simulink model "plant_block"  (R2025b)
settings: Solver=VariableStepAuto  StartTime=0.0  StopTime=10.0  RelTol=1e-3
undefined symbols (not defined in the file): auv
settings Model: Creator=Heisenberg  LastModifiedBy=Heisenberg

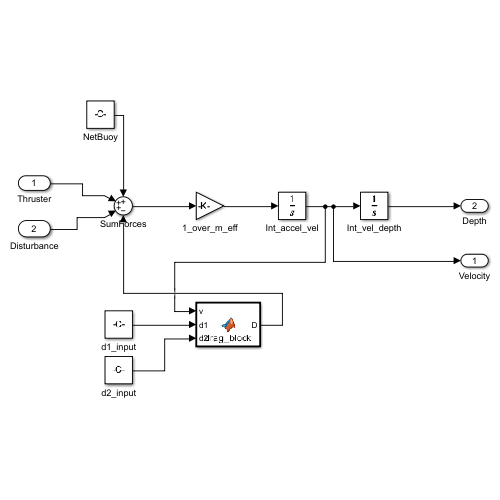
[thumbnail: Simulink's stored preview of the top-level diagram]
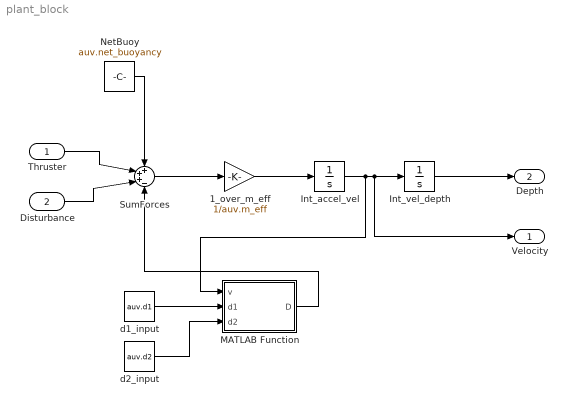
== system plant_block ==
  Thruster : Inport
  Disturbance : Inport  Port=2
  1_over_m_eff : Gain  Gain=1/auv.m_eff
  Int_accel_vel : Integrator
  Int_vel_depth : Integrator
  MATLAB Function : MATLAB Function  TreatAsAtomicUnit=on
  NetBuoy : Constant  Value=auv.net_buoyancy
  SumForces : Sum  Inputs=+++-
  d1_input : Constant  Value=auv.d1
  d2_input : Constant  Value=auv.d2
  Velocity : Outport
  Depth : Outport  Port=2
  wires:
  NetBuoy/1 -> SumForces/1
  SumForces/1 -> 1_over_m_eff/1
  1_over_m_eff/1 -> Int_accel_vel/1
  MATLAB Function/1(D) -> SumForces/4
  Int_accel_vel/1 -> MATLAB Function/1(v), Velocity/1, Int_vel_depth/1
  Thruster/1 -> SumForces/2
  Disturbance/1 -> SumForces/3
  Int_vel_depth/1 -> Depth/1
  d1_input/1 -> MATLAB Function/2(d1)
  d2_input/1 -> MATLAB Function/3(d2)

== matlab function plant_block/MATLAB Function ==
  data: v input; D output; d1 input; d2 input
function D = drag_block(v, d1, d2)
% v : velocity
% d1, d2 : drag coefficients

D = d1 * v + d2 * abs(v).*v;
end
